simulink library "Scene_Utilities"  (R2024b)
settings: Solver=VariableStepAuto  StartTime=0.0  StopTime=10.0  RelTol=1e-3
undefined symbols (not defined in the file): circ_out, RDF_Rough_Road, X, Y, Z
libraries: sm_lib x76, $bdroot x52, Multibody_Parts_Lib x2
(part 1 of 3)
Description:
  | Simscape Vehicle Templates Library
  | 
  | Copyright 2018-2024 The MathWorks, Inc.
settings Model: Creator=smiller  LastModifiedBy=smiller
settings ModelReferenceCC: EnableRefExpFcnMdlSchedulingChecks=on
settings RTWCC: GPUComputeCapability=3.5

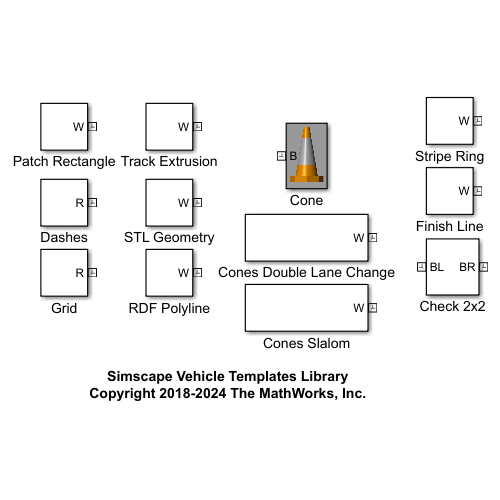
[thumbnail: Simulink's stored preview of the top-level diagram]
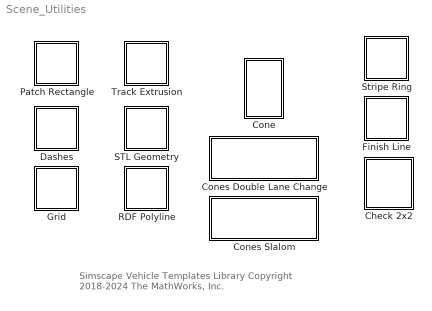
== system Scene_Utilities ==
  note: Simscape Vehicle Templates Library
      | Copyright 2018-2024 The MathWorks, Inc.
  Check 2x2 : Subsystem  mask{square_lwh=[0.01 1 1]}
      mask prompts: square_lwh "Size [l w h] (m)"
  Cone : Subsystem  mask(Cone){height=1, baseThickness=0.1, baseWidth=0.6, coneBaseDiameter=0.4, coneTopDiameter=0.1, reflectiveStripHeight=0.5, opc=1, coneColor=[1 0.6 0], reflectiveStripColor=[0.75 0.75 0.75]}
      mask prompts: height "Height (m)"; baseThickness "Base Thickness (m)"; baseWidth "Base Width (m)"; coneBaseDiameter "Cone Base Diameter (m)"; coneTopDiameter "Cone Top Diameter (m)"; reflectiveStripHeight "Reflective Strip Height (m)"; opc "Opacity"; coneColor "Cone Color [r g b]"; reflectiveStripColor "Reflective Strip Color [r g b]"
      mask help:
      | This block models a traffic cone. The block comprises an octagonal base with a conical upper.
      |
      | Port B corresponds to the center point of the bottom surface of the base with the z-axis aligned with the conical axis.
      mask init:
      | coneBaseHeight = 0.5 * (height - baseThickness - reflectiveStripHeight);
      | 
      | coneHeight = height - baseThickness;
      | 
      | coneBaseRadius = 0.5 * coneBaseDiameter;
      | coneTopRadius2 = 0.5 * coneTopDiameter;
      | 
      | coneRadDiff = coneBaseRadius - coneTopRadius2;
      | 
      | coneBaseRadius2 = coneBaseRadius - coneBaseHeight * coneRadDiff / coneHeight;
      | 
      | coneBaseCrossSection = [0 0; 
      |                         coneBaseRadius 0;
      |                         coneBaseRadius2 coneBaseHeight;
      |                         0 coneBaseHeight];
      | 
      | coneTopHeight = coneBaseHeight;
      | coneTopRadius1 = coneTopRadius2 + coneTopHeight * coneRadDiff / coneHeight;
      |                       
      | reflectiveStripCrossSection = [0 0;
      |                                coneBaseRadius2 0;
      |                                coneTopRadius1 reflectiveStripHeight;
      |                                0 reflectiveStripHeight];
      |                              
      | coneTopCrossSection = [0 0;
      |                        coneTopRadius1 0;
      |                        coneTopRadius2 coneTopHeight;
      |                        0 coneTopHeight];
      mask DialogControl Tab1 Prompt: Dimensions
      mask DialogControl Tab2 Prompt: Material Properties
      mask Display: image('sm_vehicle_slalom_cone.png');
  Cones Double Lane Change : Subsystem  mask{lane_width=3.3, lane_separation=4.1, start_lane_a=173.8, A1_to_A5=12.5, A_to_B_x=12.7, B1_to_B5=12.3, B_to_C_x=12.7, C1_to_C5=12, height=0.6, baseThickness=0.04, baseWidth=0.5, coneBaseDiameter=0.24, coneTopDiameter=0.06, reflectiveStripHeight=0.3, coneColor=[248 78 25]/255, reflectiveStripColor=[0.75 0.75 0.75]}
      mask prompts: lane_width "Lane Width (m)"; lane_separation "Lane Lateral Separation (m)"; start_lane_a "Distance to start Lane A (m)"; A1_to_A5 "Distance Cone 1 to 5 (m) Lane A"; A_to_B_x "Distance Lane A to Lane B (m)"; B1_to_B5 "Distance Cone 1 to 5 (m) Lane B"; B_to_C_x "Distance Lane B to Lane C (m)"; C1_to_C5 "Distance Cone 1 to 5 (m) Lane C"; height "Height (m)"; baseThickness "Base Thickness (m)"; baseWidth "Base Width (m)"; coneBaseDiameter "Cone Base Diameter (m)"; coneTopDiameter "Cone Top Diameter (m)"; reflectiveStripHeight "Reflective Strip Height (m)"; coneColor "Cone Color [RGB]"; reflectiveStripColor "Reflective Strip Color [RGB]"
      mask DialogControl cont_placement Prompt: Placement
      mask DialogControl cont_appearance Prompt: Appearance
  Cones Slalom : Subsystem  mask{y_cones=4.1, x_cone_1=173.8, x_cone_spacing=12.5, num_cones=5, height=0.6, baseThickness=0.04, baseWidth=0.5, coneBaseDiameter=0.24, coneTopDiameter=0.06, reflectiveStripHeight=0.3, coneColor=[248 78 25]/255, reflectiveStripColor=[0.75 0.75 0.75]}
      mask prompts: y_cones "Lateral Offset (m)"; x_cone_1 "Longitudinal Distance to Cone 1 (m)"; x_cone_spacing "Distance Between Cones"; num_cones "Number of Cones"; height "Height (m)"; baseThickness "Base Thickness (m)"; baseWidth "Base Width (m)"; coneBaseDiameter "Cone Base Diameter (m)"; coneTopDiameter "Cone Top Diameter (m)"; reflectiveStripHeight "Reflective Strip Height (m)"; coneColor "Cone Color [RGB]"; reflectiveStripColor "Reflective Strip Color [RGB]"
      mask init:
      | visCones = ones(1,num_cones);
      | hidCones = zeros(1,12-num_cones);
      | opcvec   = [visCones hidCones];
      mask DialogControl cont_placement Prompt: Placement
      mask DialogControl cont_appearance Prompt: Appearance
  Dashes : Subsystem  mask{dash_pitch=7.5, num_dashes=4, dash_l=3, dash_h=2, dash_w=0.15, thickness_base=4, dash_clr=[1 1 1], dash_opc=1}
      mask prompts: dash_pitch "Distance between dash centers (m)"; num_dashes "Number of dashes"; dash_l "Dash length (m)"; dash_h "Dash height (m)"; dash_w "Dash width (m)"; thickness_base "Height base of solid (m)"; dash_clr "Color [RGB]"; dash_opc "Opacity (0-1)"
      mask init:
      | dash_extr_data = Extr_Data_Dashes(dash_pitch,num_dashes,dash_l,dash_h,thickness_base);
  Finish Line : Subsystem  mask{post_h=6, post_r=0.5, line_w=18, post_clr=[0.8 0.0 0.2], post_opc=1, offset_xyz=[0 0 0], offset_yaw=0, offset_pitch=0, offset_roll=0}
      mask prompts: post_h "Post Height (m)"; post_r "Post Radius (m)"; line_w "Post Separation (m)"; post_clr "Post Color [R G B] (0-1)"; post_opc "Post Opacity (0-1)"; offset_xyz "Line Offset [x y z] (m)"; offset_yaw "Line Orientation yaw (rad)"; offset_pitch "Line Orientation pitch (rad)"; offset_roll "Line Orientation roll (rad)"
  Grid : Subsystem  mask{grid_x=400, grid_y=400, grid_z=0.02, grid_line_width=0.08, grid_num_sq_x=10, grid_num_sq_y=17, grid_clr=[1 1 1], grid_opc=1}
      mask prompts: grid_x "Length (m) (Global x)"; grid_y "Width (m) (Global y)"; grid_z "Depth (m) (Global z)"; grid_line_width "Line width (m)"; grid_num_sq_x "Number of squares in x"; grid_num_sq_y "Number of squares in y"; grid_clr "Color [RGB]"; grid_opc "Opacity (0-1)"
      mask init:
      | % Derived parameters - for two perpendicular grids with num_sq-by-1 holes
      | % **Note, not num_sq_x by num_sq_y holes - better render speed with
      | % separate meshes for x and y.
      | 
      | hole_lx = (grid_x-(grid_line_width*(grid_num_sq_x+1)))/grid_num_sq_x;
      | hole_wx = (grid_y-(grid_line_width*(1+1)))/1;
      | 
      | hole_ly = (grid_y-(grid_line_width*(grid_num_sq_y+1)))/grid_num_sq_y;
      | hole_wy = (grid_x-(grid_line_width*(1+1)))/1;
  Patch Rectangle : Subsystem  mask{gp_l=400, gp_w=400, gp_h=0.01, gp_clr=[0.8000 0.8000 0.8000], gp_opc=1}
      mask prompts: gp_l "Length (m) (Global  x)"; gp_w "Width (m) (Global  y)"; gp_h "Depth (m) (Global z)"; gp_clr "Color [R G B]"; gp_opc "Opacity (0-1)"
  RDF Polyline : Subsystem  mask{road_extr_data_L=RDF_Rough_Road.Road.extr_data_L, road_extr_data_R=RDF_Rough_Road.Road.extr_data_R, road_profile_sep=RDF_Rough_Road.Road.profile_separation, road_w=RDF_Rough_Road.Road.w, road_x=RDF_Rough_Road.Road.x, road_z=RDF_Rough_Road.Road.z, road_yaw=RDF_Rough_Road.Road.yaw, road_clr=RDF_Rough_Road.Road.clr, road_opc=RDF_Rough_Road.Road.opc}
      mask prompts: road_extr_data_L "Road Profile Left [x y] (m)"; road_extr_data_R "Road Profile Right [x y] (m)"; road_profile_sep "Profile Separation (m)"; road_w "Width (m)"; road_x "Offset x (m)"; road_z "Offset z (m)"; road_yaw "Offset yaw (rad)"; road_clr "Color [R G B]"; road_opc "Opacity (0-1)"
  STL Geometry : Subsystem  mask{stl_file='Bar1_Default_sldprt.STL', stl_units='m', stl_clr=[0.8000 0.8000 0.8000], stl_opc=1, stl_x=0, stl_y=0, stl_z=0, stl_yaw=0, stl_pitch=0, stl_roll=0}
      mask prompts: stl_file "CAD File"; stl_units "Units"; stl_clr "Color [R G B]"; stl_opc "Opacity (0-1)"; stl_x "Offset x (m)"; stl_y "Offset y (m)"; stl_z "Offset z (m)"; stl_yaw "Offset yaw (rad)"; stl_pitch "Offset pitch (rad)"; stl_roll "Offset roll (rad)"
      mask init:
      | set_param([gcb '/Geometry'],'ExtGeomFileName',stl_file);
      | set_param([gcb '/Geometry'],'ExtGeomFileUnits',stl_units);
  Stripe Ring : Subsystem  mask{circ_d=circ_out.d, circ_a1=circ_out.ang1, circ_a2=circ_out.ang2, circ_w=circ_out.w, circ_h=circ_out.h, circ_clr=circ_out.clr, circ_opc=circ_out.opc}
      mask prompts: circ_d "Circle Diameter (m)"; circ_a1 "Start Angle (deg)"; circ_a2 "Finish Angle (deg)"; circ_w "Stripe Width (m)"; circ_h "Stripe Height (m)"; circ_clr "Color [RGB]"; circ_opc "Opacity (0-1)"
      mask init:
      | xy_data_circ = Extr_Data_Ring(...
      |     circ_d/2+circ_w/2,circ_d/2-circ_w/2,circ_a1, circ_a2);
  Track Extrusion : Subsystem  mask{track_ctrline=[sin(0:0.1:(2*pi-0.1))' cos(0:0.1:(2*pi-0.1))' cos(0:0.1:(2*pi-0.1))']*10, track_w=2, track_h=0.1, track_x=0, track_y=0, track_z=0, track_yaw=0, track_clr=[0.8000 0.8000 0.8000], track_opc=1}
      mask prompts: track_ctrline "Centerline profile [x y] (m)"; track_w "Width (m)"; track_h "Height (m)"; track_x "Offset x (m)"; track_y "Offset y (m)"; track_z "Offset z (m)"; track_yaw "Offset yaw (rad)"; track_clr "Color [R G B]"; track_opc "Opacity (0-1)"
      mask init:
      | track_extr_data = sm_car_road_track_extrusion(track_ctrline,track_w);

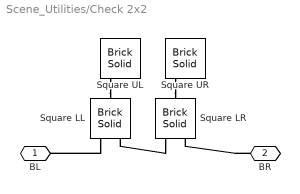
== system Scene_Utilities/Check 2x2 ==
  Square LL : sm_lib/Body Elements/Brick Solid  BrickDimensions=square_lwh  BrickDimensionsUnits=m  ExportEntireGeometry=off  InertiaType=CalculateFromGeometry  BasedOnType=Density  Density=1000  DensityUnits=kg/m^3  Mass=1  MassUnits=kg  CenterOfMass=[0 0 0]  CenterOfMassUnits=m  MomentsOfInertia=[1 1 1]  MomentsOfInertiaUnits=kg*m^2  ProductsOfInertia=[0 0 0]  ProductsOfInertiaUnits=kg*m^2  GraphicType=FromGeometry  MarkerShape=Sphere  MarkerSize=10  GraphicVisPropType=SimpleVisualProperties  GraphicDiffuseColor=[0.0 0.0 0.0]  GraphicOpacity=1.0  GraphicSpecularColor=[0.5 0.5 0.5 1.0]  GraphicAmbientColor=[0.15 0.15 0.15 1.0]  GraphicEmissiveColor=[0.0 0.0 0.0 1.0]  GraphicShininess=75  DoExposeReferenceFrame=off  SerializedFrames=<Frames><Frame><Id>Frame1</Id><Value><Name>BL</Name><Origin><Source>GeometricFeature</Source><FeatureName>+y -z curve</FeatureName></Origin><PrimaryAxis><DefinedDirection>+Z</DefinedDirection><Source>ReferenceFrame</Source><SourceDirection>+Z</SourceDirection><FeatureName></FeatureName></PrimaryAxis><SecondaryAxis><DefinedDirection>+X</DefinedDirection><Source>ReferenceFrame</Source><SourceDirection>+X</SourceDirection><FeatureName></FeatureName></SecondaryAxis></Value></Frame><Frame><Id>Frame2</Id><Value><Name>TL</Name><Origin><Source>GeometricFeature</Source><FeatureName>+x +y +z point</FeatureName></Origin><PrimaryAxis><DefinedDirection>+Z</DefinedDirection><Source>ReferenceFrame</Source><SourceDirection>+Z</SourceDirection><FeatureName></FeatureName></PrimaryAxis><SecondaryAxis><DefinedDirection>+X</DefinedDirection><Source>ReferenceFrame</Source><SourceDirection>+X</SourceDirection><FeatureName></FeatureName></SecondaryAxis></Value></Frame><Frame><Id>Frame3</Id><Value><Name>BR</Name><Origin><Source>GeometricFeature</Source><FeatureName>-y -z curve</FeatureName></Origin><PrimaryAxis><DefinedDirection>+Z</DefinedDirection><Source>ReferenceFrame</Source><SourceDirection>+Z</SourceDirection><FeatureName></FeatureName></PrimaryAxis><SecondaryAxis><DefinedDirection>+X</DefinedDirection><Source>ReferenceFrame</Source><SourceDirection>+X</SourceDirection><FeatureName></FeatureName></SecondaryAxis></Value></Frame></Frames>
  Square LR : sm_lib/Body Elements/Brick Solid  BrickDimensions=square_lwh  BrickDimensionsUnits=m  ExportEntireGeometry=off  InertiaType=CalculateFromGeometry  BasedOnType=Density  Density=1000  DensityUnits=kg/m^3  Mass=1  MassUnits=kg  CenterOfMass=[0 0 0]  CenterOfMassUnits=m  MomentsOfInertia=[1 1 1]  MomentsOfInertiaUnits=kg*m^2  ProductsOfInertia=[0 0 0]  ProductsOfInertiaUnits=kg*m^2  GraphicType=FromGeometry  MarkerShape=Sphere  MarkerSize=10  GraphicVisPropType=SimpleVisualProperties  GraphicDiffuseColor=[1.0 1.0 1.0]  GraphicOpacity=1.0  GraphicSpecularColor=[0.5 0.5 0.5 1.0]  GraphicAmbientColor=[0.15 0.15 0.15 1.0]  GraphicEmissiveColor=[0.0 0.0 0.0 1.0]  GraphicShininess=75  DoExposeReferenceFrame=off  SerializedFrames=<Frames><Frame><Id>Frame1</Id><Value><Name>BL</Name><Origin><Source>GeometricFeature</Source><FeatureName>+y -z curve</FeatureName></Origin><PrimaryAxis><DefinedDirection>+Z</DefinedDirection><Source>ReferenceFrame</Source><SourceDirection>+Z</SourceDirection><FeatureName></FeatureName></PrimaryAxis><SecondaryAxis><DefinedDirection>+X</DefinedDirection><Source>ReferenceFrame</Source><SourceDirection>+X</SourceDirection><FeatureName></FeatureName></SecondaryAxis></Value></Frame><Frame><Id>Frame2</Id><Value><Name>TL</Name><Origin><Source>GeometricFeature</Source><FeatureName>+x +y +z point</FeatureName></Origin><PrimaryAxis><DefinedDirection>+Z</DefinedDirection><Source>ReferenceFrame</Source><SourceDirection>+Z</SourceDirection><FeatureName></FeatureName></PrimaryAxis><SecondaryAxis><DefinedDirection>+X</DefinedDirection><Source>ReferenceFrame</Source><SourceDirection>+X</SourceDirection><FeatureName></FeatureName></SecondaryAxis></Value></Frame><Frame><Id>Frame3</Id><Value><Name>BR</Name><Origin><Source>GeometricFeature</Source><FeatureName>-y -z curve</FeatureName></Origin><PrimaryAxis><DefinedDirection>+Z</DefinedDirection><Source>ReferenceFrame</Source><SourceDirection>+Z</SourceDirection><FeatureName></FeatureName></PrimaryAxis><SecondaryAxis><DefinedDirection>+X</DefinedDirection><Source>ReferenceFrame</Source><SourceDirection>+X</SourceDirection><FeatureName></FeatureName></SecondaryAxis></Value></Frame></Frames>
  Square UL : sm_lib/Body Elements/Brick Solid  BrickDimensions=square_lwh  BrickDimensionsUnits=m  ExportEntireGeometry=off  InertiaType=CalculateFromGeometry  BasedOnType=Density  Density=1000  DensityUnits=kg/m^3  Mass=1  MassUnits=kg  CenterOfMass=[0 0 0]  CenterOfMassUnits=m  MomentsOfInertia=[1 1 1]  MomentsOfInertiaUnits=kg*m^2  ProductsOfInertia=[0 0 0]  ProductsOfInertiaUnits=kg*m^2  GraphicType=FromGeometry  MarkerShape=Sphere  MarkerSize=10  GraphicVisPropType=SimpleVisualProperties  GraphicDiffuseColor=[1.0 1.0 1.0]  GraphicOpacity=1.0  GraphicSpecularColor=[0.5 0.5 0.5 1.0]  GraphicAmbientColor=[0.15 0.15 0.15 1.0]  GraphicEmissiveColor=[0.0 0.0 0.0 1.0]  GraphicShininess=75  DoExposeReferenceFrame=off  SerializedFrames=<Frames><Frame><Id>Frame1</Id><Value><Name>BL</Name><Origin><Source>GeometricFeature</Source><FeatureName>+y -z curve</FeatureName></Origin><PrimaryAxis><DefinedDirection>+Z</DefinedDirection><Source>ReferenceFrame</Source><SourceDirection>+Z</SourceDirection><FeatureName></FeatureName></PrimaryAxis><SecondaryAxis><DefinedDirection>+X</DefinedDirection><Source>ReferenceFrame</Source><SourceDirection>+X</SourceDirection><FeatureName></FeatureName></SecondaryAxis></Value></Frame><Frame><Id>Frame2</Id><Value><Name>TL</Name><Origin><Source>GeometricFeature</Source><FeatureName>+x +y +z point</FeatureName></Origin><PrimaryAxis><DefinedDirection>+Z</DefinedDirection><Source>ReferenceFrame</Source><SourceDirection>+Z</SourceDirection><FeatureName></FeatureName></PrimaryAxis><SecondaryAxis><DefinedDirection>+X</DefinedDirection><Source>ReferenceFrame</Source><SourceDirection>+X</SourceDirection><FeatureName></FeatureName></SecondaryAxis></Value></Frame><Frame><Id>Frame3</Id><Value><Name>BR</Name><Origin><Source>GeometricFeature</Source><FeatureName>-y -z curve</FeatureName></Origin><PrimaryAxis><DefinedDirection>+Z</DefinedDirection><Source>ReferenceFrame</Source><SourceDirection>+Z</SourceDirection><FeatureName></FeatureName></PrimaryAxis><SecondaryAxis><DefinedDirection>+X</DefinedDirection><Source>ReferenceFrame</Source><SourceDirection>+X</SourceDirection><FeatureName></FeatureName></SecondaryAxis></Value></Frame></Frames>
  Square UR : sm_lib/Body Elements/Brick Solid  BrickDimensions=square_lwh  BrickDimensionsUnits=m  ExportEntireGeometry=off  InertiaType=CalculateFromGeometry  BasedOnType=Density  Density=1000  DensityUnits=kg/m^3  Mass=1  MassUnits=kg  CenterOfMass=[0 0 0]  CenterOfMassUnits=m  MomentsOfInertia=[1 1 1]  MomentsOfInertiaUnits=kg*m^2  ProductsOfInertia=[0 0 0]  ProductsOfInertiaUnits=kg*m^2  GraphicType=FromGeometry  MarkerShape=Sphere  MarkerSize=10  GraphicVisPropType=SimpleVisualProperties  GraphicDiffuseColor=[0.0 0.0 0.0]  GraphicOpacity=1.0  GraphicSpecularColor=[0.5 0.5 0.5 1.0]  GraphicAmbientColor=[0.15 0.15 0.15 1.0]  GraphicEmissiveColor=[0.0 0.0 0.0 1.0]  GraphicShininess=75  DoExposeReferenceFrame=off  SerializedFrames=<Frames><Frame><Id>Frame1</Id><Value><Name>BL</Name><Origin><Source>GeometricFeature</Source><FeatureName>+y -z curve</FeatureName></Origin><PrimaryAxis><DefinedDirection>+Z</DefinedDirection><Source>ReferenceFrame</Source><SourceDirection>+Z</SourceDirection><FeatureName></FeatureName></PrimaryAxis><SecondaryAxis><DefinedDirection>+X</DefinedDirection><Source>ReferenceFrame</Source><SourceDirection>+X</SourceDirection><FeatureName></FeatureName></SecondaryAxis></Value></Frame><Frame><Id>Frame2</Id><Value><Name>TL</Name><Origin><Source>GeometricFeature</Source><FeatureName>+x +y +z point</FeatureName></Origin><PrimaryAxis><DefinedDirection>+Z</DefinedDirection><Source>ReferenceFrame</Source><SourceDirection>+Z</SourceDirection><FeatureName></FeatureName></PrimaryAxis><SecondaryAxis><DefinedDirection>+X</DefinedDirection><Source>ReferenceFrame</Source><SourceDirection>+X</SourceDirection><FeatureName></FeatureName></SecondaryAxis></Value></Frame><Frame><Id>Frame3</Id><Value><Name>BR</Name><Origin><Source>GeometricFeature</Source><FeatureName>-y -z curve</FeatureName></Origin><PrimaryAxis><DefinedDirection>+Z</DefinedDirection><Source>ReferenceFrame</Source><SourceDirection>+Z</SourceDirection><FeatureName></FeatureName></PrimaryAxis><SecondaryAxis><DefinedDirection>+X</DefinedDirection><Source>ReferenceFrame</Source><SourceDirection>+X</SourceDirection><FeatureName></FeatureName></SecondaryAxis></Value></Frame></Frames>
  BL : PMIOPort  Side=Left
  BR : PMIOPort  Port=2  Side=Right
  connections:
  BR/RConn1 -- Square LR/LConn2
  Square UR/LConn1 -- Square LR/RConn1
  Square UL/LConn1 -- Square LL/RConn1
  Square LL/LConn1 -- BL/RConn1
  Square LR/LConn1 -- Square LL/LConn2

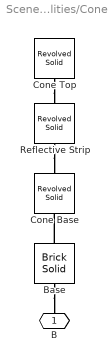
== system Scene_Utilities/Cone ==
  Base : sm_lib/Body Elements/Brick Solid  BrickDimensions=[baseWidth baseWidth baseThickness]  BrickDimensionsUnits=m  ExportEntireGeometry=off  InertiaType=CalculateFromGeometry  BasedOnType=Density  Density=1000  DensityUnits=kg/m^3  Mass=1  MassUnits=kg  CenterOfMass=[0 0 0]  CenterOfMassUnits=m  MomentsOfInertia=[1 1 1]  MomentsOfInertiaUnits=kg*m^2  ProductsOfInertia=[0 0 0]  ProductsOfInertiaUnits=kg*m^2  GraphicType=FromGeometry  MarkerShape=Sphere  MarkerSize=10  GraphicVisPropType=SimpleVisualProperties  GraphicDiffuseColor=coneColor  GraphicOpacity=opc  GraphicSpecularColor=[0.5 0.5 0.5 1.0]  GraphicAmbientColor=[0.15 0.15 0.15 1.0]  GraphicEmissiveColor=[0.0 0.0 0.0 1.0]  GraphicShininess=75  DoExposeReferenceFrame=off  SerializedFrames=<Frames><Frame><Id>Frame1</Id><Value><Name>B</Name><Origin><Source>GeometricFeature</Source><FeatureName>-z surface</FeatureName></Origin><PrimaryAxis><DefinedDirection>+Z</DefinedDirection><Source>ReferenceFrame</Source><SourceDirection>+Z</SourceDirection><FeatureName></FeatureName></PrimaryAxis><SecondaryAxis><DefinedDirection>+X</DefinedDirection><Source>ReferenceFrame</Source><SourceDirection>+X</SourceDirection><FeatureName></FeatureName></SecondaryAxis></Value></Frame><Frame><Id>Frame2</Id><Value><Name>F</Name><Origin><Source>GeometricFeature</Source><FeatureName>+z surface</FeatureName></Origin><PrimaryAxis><DefinedDirection>+Z</DefinedDirection><Source>ReferenceFrame</Source><SourceDirection>+Z</SourceDirection><FeatureName></FeatureName></PrimaryAxis><SecondaryAxis><DefinedDirection>+X</DefinedDirection><Source>ReferenceFrame</Source><SourceDirection>+X</SourceDirection><FeatureName></FeatureName></SecondaryAxis></Value></Frame></Frames>
  Cone Base : sm_lib/Body Elements/Revolved Solid  RevolutionCrossSection=coneBaseCrossSection  RevolutionCrossSectionUnits=m  RevolutionExtent=Full  RevolutionAngle=180  RevolutionAngleUnits=deg  ExportConvexHullGeometry=off  InertiaType=CalculateFromGeometry  BasedOnType=Density  Density=1000  DensityUnits=kg/m^3  Mass=1  MassUnits=kg  CenterOfMass=[0 0 0]  CenterOfMassUnits=m  MomentsOfInertia=[1 1 1]  MomentsOfInertiaUnits=kg*m^2  ProductsOfInertia=[0 0 0]  ProductsOfInertiaUnits=kg*m^2  GraphicType=FromGeometry  MarkerShape=Sphere  MarkerSize=10  GraphicVisPropType=SimpleVisualProperties  GraphicDiffuseColor=coneColor  GraphicOpacity=opc  GraphicSpecularColor=[0.5 0.5 0.5 1.0]  GraphicAmbientColor=[0.15 0.15 0.15 1.0]  GraphicEmissiveColor=[0.0 0.0 0.0 1.0]  GraphicShininess=75  DoExposeReferenceFrame=off  SerializedFrames=<Frames><Frame><Id>Frame1</Id><Value><Name>B</Name><Origin><Source>GeometricFeature</Source><FeatureName>side surface 1</FeatureName></Origin><PrimaryAxis><DefinedDirection>+Z</DefinedDirection><Source>ReferenceFrame</Source><SourceDirection>+Z</SourceDirection><FeatureName></FeatureName></PrimaryAxis><SecondaryAxis><DefinedDirection>+X</DefinedDirection><Source>ReferenceFrame</Source><SourceDirection>+X</SourceDirection><FeatureName></FeatureName></SecondaryAxis></Value></Frame><Frame><Id>Frame2</Id><Value><Name>F</Name><Origin><Source>GeometricFeature</Source><FeatureName>side surface 3</FeatureName></Origin><PrimaryAxis><DefinedDirection>+Z</DefinedDirection><Source>ReferenceFrame</Source><SourceDirection>+Z</SourceDirection><FeatureName></FeatureName></PrimaryAxis><SecondaryAxis><DefinedDirection>+X</DefinedDirection><Source>ReferenceFrame</Source><SourceDirection>+X</SourceDirection><FeatureName></FeatureName></SecondaryAxis></Value></Frame></Frames>
  Cone Top : sm_lib/Body Elements/Revolved Solid  RevolutionCrossSection=coneTopCrossSection  RevolutionCrossSectionUnits=m  RevolutionExtent=Full  RevolutionAngle=180  RevolutionAngleUnits=deg  ExportConvexHullGeometry=off  InertiaType=CalculateFromGeometry  BasedOnType=Density  Density=1000  DensityUnits=kg/m^3  Mass=1  MassUnits=kg  CenterOfMass=[0 0 0]  CenterOfMassUnits=m  MomentsOfInertia=[1 1 1]  MomentsOfInertiaUnits=kg*m^2  ProductsOfInertia=[0 0 0]  ProductsOfInertiaUnits=kg*m^2  GraphicType=FromGeometry  MarkerShape=Sphere  MarkerSize=10  GraphicVisPropType=SimpleVisualProperties  GraphicDiffuseColor=coneColor  GraphicOpacity=opc  GraphicSpecularColor=[0.5 0.5 0.5 1.0]  GraphicAmbientColor=[0.15 0.15 0.15 1.0]  GraphicEmissiveColor=[0.0 0.0 0.0 1.0]  GraphicShininess=75  DoExposeReferenceFrame=off  SerializedFrames=<Frames><Frame><Id>Frame1</Id><Value><Name>B</Name><Origin><Source>GeometricFeature</Source><FeatureName>side surface 1</FeatureName></Origin><PrimaryAxis><DefinedDirection>+Z</DefinedDirection><Source>ReferenceFrame</Source><SourceDirection>+Z</SourceDirection><FeatureName></FeatureName></PrimaryAxis><SecondaryAxis><DefinedDirection>+X</DefinedDirection><Source>ReferenceFrame</Source><SourceDirection>+X</SourceDirection><FeatureName></FeatureName></SecondaryAxis></Value></Frame></Frames>
  Reflective Strip : sm_lib/Body Elements/Revolved Solid  RevolutionCrossSection=reflectiveStripCrossSection  RevolutionCrossSectionUnits=m  RevolutionExtent=Full  RevolutionAngle=180  RevolutionAngleUnits=deg  ExportConvexHullGeometry=off  InertiaType=CalculateFromGeometry  BasedOnType=Density  Density=1000  DensityUnits=kg/m^3  Mass=1  MassUnits=kg  CenterOfMass=[0 0 0]  CenterOfMassUnits=m  MomentsOfInertia=[1 1 1]  MomentsOfInertiaUnits=kg*m^2  ProductsOfInertia=[0 0 0]  ProductsOfInertiaUnits=kg*m^2  GraphicType=FromGeometry  MarkerShape=Sphere  MarkerSize=10  GraphicVisPropType=SimpleVisualProperties  GraphicDiffuseColor=reflectiveStripColor  GraphicOpacity=opc  GraphicSpecularColor=[0.5 0.5 0.5 1.0]  GraphicAmbientColor=[0.15 0.15 0.15 1.0]  GraphicEmissiveColor=[0.0 0.0 0.0 1.0]  GraphicShininess=75  DoExposeReferenceFrame=off  SerializedFrames=<Frames><Frame><Id>Frame1</Id><Value><Name>B</Name><Origin><Source>GeometricFeature</Source><FeatureName>side surface 1</FeatureName></Origin><PrimaryAxis><DefinedDirection>+Z</DefinedDirection><Source>ReferenceFrame</Source><SourceDirection>+Z</SourceDirection><FeatureName></FeatureName></PrimaryAxis><SecondaryAxis><DefinedDirection>+X</DefinedDirection><Source>ReferenceFrame</Source><SourceDirection>+X</SourceDirection><FeatureName></FeatureName></SecondaryAxis></Value></Frame><Frame><Id>Frame2</Id><Value><Name>F</Name><Origin><Source>GeometricFeature</Source><FeatureName>side surface 3</FeatureName></Origin><PrimaryAxis><DefinedDirection>+Z</DefinedDirection><Source>ReferenceFrame</Source><SourceDirection>+Z</SourceDirection><FeatureName></FeatureName></PrimaryAxis><SecondaryAxis><DefinedDirection>+X</DefinedDirection><Source>ReferenceFrame</Source><SourceDirection>+X</SourceDirection><FeatureName></FeatureName></SecondaryAxis></Value></Frame></Frames>
  B : PMIOPort  Side=Left
  connections:
  Base/RConn1 -- Cone Base/LConn1
  Base/LConn1 -- B/RConn1
  Cone Top/LConn1 -- Reflective Strip/RConn1
  Reflective Strip/LConn1 -- Cone Base/RConn1
